simulink model "tb_per_tebvfh"  (R2026b)
model workspace (MAT data in the model file):
  tebRefPath = [0  0  0; 5  0  0; 10  0  0; 15  0  0; 20  0  0]
undefined symbols (not defined in the file or in its folder): Ts
libraries: navlib x1, robotalgslib x1
settings Model: Creator=aomar  LastModifiedBy=aomar

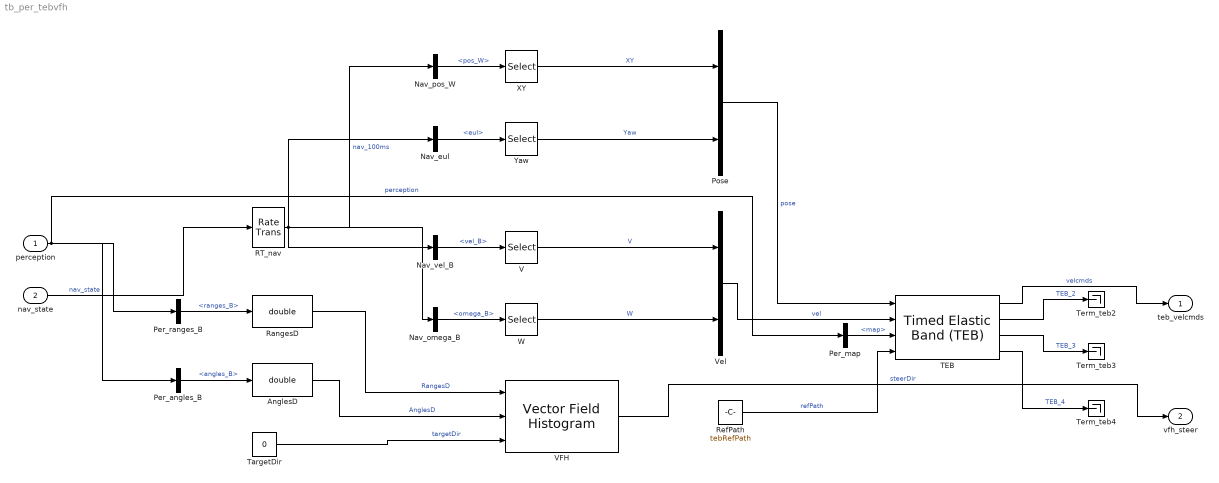
== system tb_per_tebvfh ==
  perception : Inport  OutDataTypeStr=Bus: Bus_Perception  SampleTime=Ts.perception  Interpolate=off  BusOutputAsStruct=on
  nav_state : Inport  Port=2  OutDataTypeStr=Bus: Bus_NavState  SampleTime=Ts.nav  Interpolate=off  BusOutputAsStruct=on
  AnglesD : DataTypeConversion  OutDataTypeStr=double  SaturateOnIntegerOverflow=off  RndMeth=Floor
  Nav_eul : BusSelector  OutputSignals=eul
  Nav_omega_B : BusSelector  OutputSignals=omega_B
  Nav_pos_W : BusSelector  OutputSignals=pos_W
  Nav_vel_B : BusSelector  OutputSignals=vel_B
  Per_angles_B : BusSelector  OutputSignals=angles_B
  Per_map : BusSelector  OutputSignals=map
  Per_ranges_B : BusSelector  OutputSignals=ranges_B
  Pose : Mux  Inputs=[2 1]
  RT_nav : RateTransition  OutPortSampleTime=Ts.perception
  RangesD : DataTypeConversion  OutDataTypeStr=double  SaturateOnIntegerOverflow=off  RndMeth=Floor
  RefPath : Constant  Value=tebRefPath  SampleTime=Ts.perception
  TEB : navlib/Control Algorithms/Timed Elastic Band (TEB)  ControlMode=Path Following with Obstacle Avoidance  SampleTime=Ts.perception  LookAheadTimePort=off  LookAheadTime=5  GoalTolerancePort=off  GoalTolerance=[ 0.1, 0.1, 0.1 ]  MaxVelocityPort=off  MaxVelocity=[ 0.8, 1.6 ]  MaxReverseVelocityPort=off  MaxReverseVelocity=NaN  MaxAccelerationPort=off  MaxAcceleration=[ 2.4, 4.8 ]  MinTurningRadiusPort=off  MinTurningRadius=0  ReferenceDeltaTimePort=off  ReferenceDeltaTime=0.3  NumIterationPort=off  NumIteration=2  TimePort=off  Time=10  SmoothnessPort=off  Smoothness=1000  ObstaclePort=off  Obstacle=50  Shape=Rectangle  Dimension=[ 1, 0.6700 ]  FixedTransform=se2  ObstacleSafetyMarginPort=off  ObstacleSafetyMargin=0.5
  TargetDir : Constant  Value=0  SampleTime=Ts.perception
  Term_teb2 : Terminator
  Term_teb3 : Terminator
  Term_teb4 : Terminator
  V : Selector  InputPortWidth=3  IndexOptions=Index vector (dialog)  Indices=1  OutputSizes=1
  VFH : robotalgslib/Vector Field Histogram  NumAngularSectors=180  DistanceLimits=[ 0.05, 2 ]  HistogramThresholds=[ 3, 10 ]  RobotRadius=0.1  SafetyDistance=0.1  MinTurningRadius=0.1  SimulateUsing=Code generation  TargetDirectionWeight=5  CurrentDirectionWeight=2  PreviousDirectionWeight=2
      settings: LibrarySourceBlock=navlib/Control Algorithms/Vector Field Histogram
  Vel : Mux  Inputs=2
  W : Selector  InputPortWidth=3  IndexOptions=Index vector (dialog)  Indices=3  OutputSizes=1
  XY : Selector  InputPortWidth=3  IndexOptions=Index vector (dialog)  Indices=[1 2]  OutputSizes=1
  Yaw : Selector  InputPortWidth=3  IndexOptions=Index vector (dialog)  Indices=1  OutputSizes=1
  teb_velcmds : Outport
  vfh_steer : Outport  Port=2
  wires:
  perception/1 -> Per_angles_B/1, Per_map/1, Per_ranges_B/1  "perception"
  nav_state/1 -> RT_nav/1  "nav_state"
  Per_ranges_B/1 -> RangesD/1  "<ranges_B>"
  Per_angles_B/1 -> AnglesD/1  "<angles_B>"
  TargetDir/1 -> VFH/3  "targetDir"
  RT_nav/1 -> Nav_pos_W/1, Nav_omega_B/1, Nav_eul/1, Nav_vel_B/1  "nav_100ms"
  RangesD/1 -> VFH/1  "RangesD"
  AnglesD/1 -> VFH/2  "AnglesD"
  Nav_pos_W/1 -> XY/1  "<pos_W>"
  Nav_eul/1 -> Yaw/1  "<eul>"
  Nav_vel_B/1 -> V/1  "<vel_B>"
  Nav_omega_B/1 -> W/1  "<omega_B>"
  XY/1 -> Pose/1  "XY"
  Yaw/1 -> Pose/2  "Yaw"
  V/1 -> Vel/1  "V"
  W/1 -> Vel/2  "W"
  VFH/1 -> vfh_steer/1  "steerDir"
  Pose/1 -> TEB/1  "pose"
  Vel/1 -> TEB/2  "vel"
  RefPath/1 -> TEB/4  "refPath"
  Per_map/1 -> TEB/3  "<map>"
  TEB/1 -> teb_velcmds/1  "velcmds"
  TEB/2 -> Term_teb2/1  "TEB_2"
  TEB/3 -> Term_teb3/1  "TEB_3"
  TEB/4 -> Term_teb4/1  "TEB_4"
